simulink model "Inverter_book"  (R2025a)
settings: Solver=VariableStepAuto  StartTime=0.0  StopTime=0.1  RelTol=1e-3
libraries: spsSeriesRLCBranchLib x5, spsCurrentMeasurementLib x4, spsDiodeLib x4, spsMosfetLib x4, spsVoltageMeasurementLib x4, spsDCVoltageSourceLib x1, spsMutualInductanceLib x1, spspowerguiLib x1
settings Model: Creator=Admin  LastModifiedBy=Athip

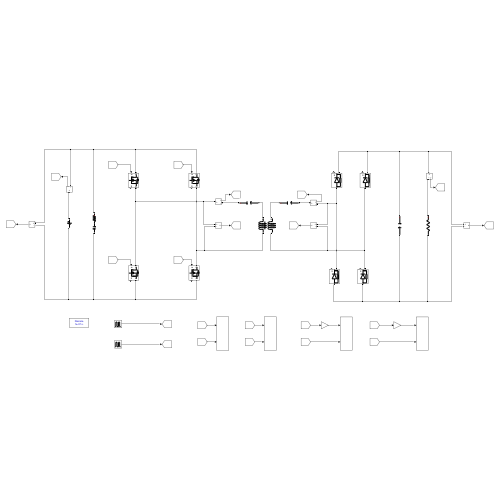
[thumbnail: Simulink's stored preview of the top-level diagram]
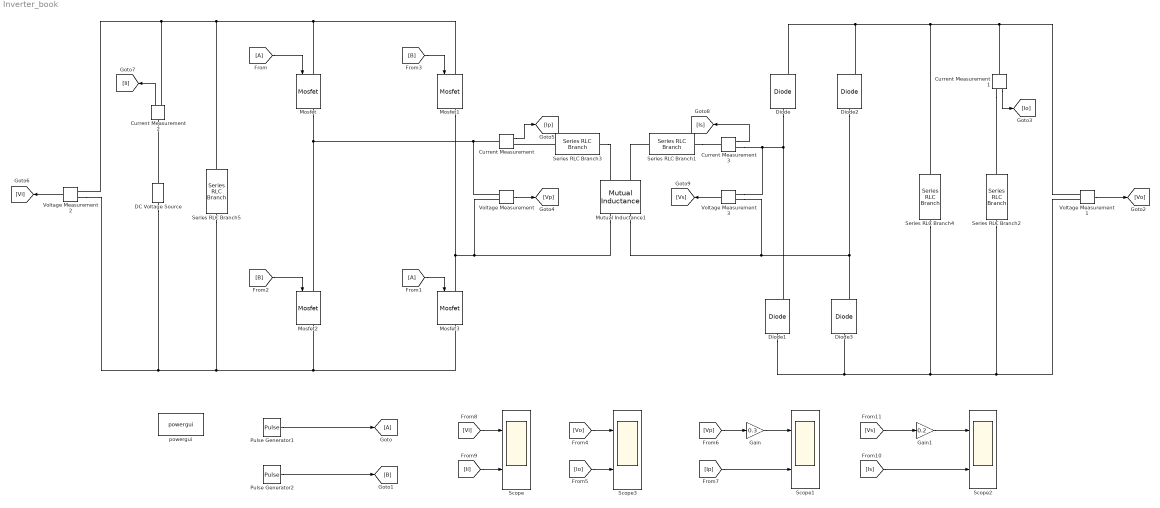
== system Inverter_book ==
  Current Measurement{,1..3} (4 alike) : spsCurrentMeasurementLib/Current Measurement  PhasorSimulation=off  OutputType=Complex  PSBequivalent=0
  DC Voltage Source : spsDCVoltageSourceLib/DC Voltage Source  Amplitude=10  Measurements=None
  Diode{,1..3} (4 alike) : spsDiodeLib/Diode  Ron=0.001  Lon=0  Vf=0.45  IC=0  UseSnubber=0  Rs=500  Cs=250e-9  Measurements=on
  From : From
  From1 : From
  Gain : Gain  Gain=0.3
  Gain1 : Gain  Gain=0.2
  Goto : Goto
  Mosfet{,1..3} (4 alike) : spsMosfetLib/Mosfet  Ron=0.0175  Lon=0  Rd=0.01  Vfd=0  IC=0  Rs=1e5  Cs=inf  Measurements=on
  Mutual Inductance1 : spsMutualInductanceLib/Mutual Inductance  LConnTagsString=a|b  RConnTagsString=A|B  TypeOfMutual=Two or three windings with equal mutual terms  NumberOfWindings=3  SelfImpedance1=[520.266e-3 16.7529e-6]  SelfImpedance2=[508.686e-3 16.0486e-6]  ThreeWindings=off  SelfImpedance3=[ 1.1 1.1e-03]  MutualImpedance=[0 7.19e-6]  InductanceMatrix="[1.0 0.9  0.9 ;  0.9 1.0  0.9;  0.9 0.9 1.0 ] * 1e-3"  ResistanceMatrix="[1.0 0.9  0.9 ;  0.9 1.0  0.9;  0.9 0.9 1.0 ]"  Measurements=None
      settings: LibrarySourceBlock=sps_lib/Passives/Mutual Inductance
  Pulse Generator1 : DiscretePulseGenerator  PulseType=Time based  Amplitude=15  Period=11.76e-6  PulseWidth=47.87
  Pulse Generator2 : DiscretePulseGenerator  PulseType=Time based  Amplitude=15  Period=11.76e-6  PulseWidth=47.87  PhaseDelay=11.76e-6/2
  Scope{,1..3} (4 alike) : Scope  NumInputPorts=2
      Scope settings: ActiveDisplayYMinimum=9  ActiveDisplayYMaximum=11
      Scope1 settings: ActiveDisplayYMinimum=-1.3979646704060489  ActiveDisplayYMaximum=4.2255749021124185
      Scope3 settings: ActiveDisplayYMinimum=0  ActiveDisplayYMaximum=18
  Series RLC Branch1 : spsSeriesRLCBranchLib/Series RLC Branch  LConnTagsString=__new0  RConnTagsString=__new0  BranchType=C  Resistance=1  Inductance=1e-3  SetiL0=off  InitialCurrent=0  Capacitance=216.1e-9  Setx0=off  InitialVoltage=0  Measurements=None
  Series RLC Branch2 : spsSeriesRLCBranchLib/Series RLC Branch  LConnTagsString=__new0  RConnTagsString=__new0  BranchType=R  Resistance=10  Inductance=1e-3  SetiL0=off  InitialCurrent=0  Capacitance=188.795e-9  Setx0=off  InitialVoltage=0  Measurements=None
  Series RLC Branch3 : spsSeriesRLCBranchLib/Series RLC Branch  LConnTagsString=__new0  RConnTagsString=__new0  BranchType=C  Resistance=1  Inductance=1e-3  SetiL0=off  InitialCurrent=0  Capacitance=214.4e-9  Setx0=off  InitialVoltage=0  Measurements=None
  Series RLC Branch4 : spsSeriesRLCBranchLib/Series RLC Branch  LConnTagsString=__new0  RConnTagsString=__new0  BranchType=C  Resistance=1  Inductance=1e-3  SetiL0=off  InitialCurrent=0  Capacitance=470e-6  Setx0=off  InitialVoltage=0  Measurements=None
  Series RLC Branch5 : spsSeriesRLCBranchLib/Series RLC Branch  LConnTagsString=__new0  RConnTagsString=__new0  BranchType=RC  Resistance=0.001  Inductance=1e-3  SetiL0=off  InitialCurrent=0  Capacitance=660e-6  Setx0=off  InitialVoltage=0  Measurements=None
  Voltage Measurement{,1..3} (4 alike) : spsVoltageMeasurementLib/Voltage Measurement  PhasorSimulation=off  OutputType=Complex  PSBequivalent=0
  powergui : spspowerguiLib/powergui  Priority=1  SimulationMode=Discrete  SampleTime=1e-7  frequency=60  Iterations=50  frequencyindice=0  Pbase=100e6  ErrMax=1e-4  UnitsV=kV  UnitsW=MW  buscounter=0  FunctionMessages=off  echomessages=off  EnableUseOfTLC=off  CurrentSourceSwitches=off  DisableSnubberDevices=off  DisableRonSwitches=off  DisableVfSwitches=off  DisplayEquations=off  AutomaticDiscreteSolvers=off  SolverType=Tustin/Backward Euler (TBE)  Interpol=off  ExternalGateDelay=off  methode=off  Ts=100  x0status=blocks  SPID=on  SwTol=0  HookPort=off  NonlinearTolerance=1e-4  nMaxIteration=100  ContinueOnMaxIteration=off  RestoreLinks=warning  ResistiveCurrentMeasurement=off  Frange=[0:2:500]  Ylog=off  Xlog=on  ShowGrid=off  save=off  variable=ZData  structure=0  ZoomFFT=off  StartTime=0.0  cycles=1  DisplayStyle=1  fundamental=60  FreqAxis=off  MaxFrequency=1000  frequencyindicesteady=1  RmsSteady=1  display=off
  wires:
  Pulse Generator1/1 -> Goto/1
  From/1 -> Mosfet/1
  From1/1 -> Mosfet3/1
  [B] -> Mosfet2/1
  [B] -> Mosfet1/1
  Voltage Measurement/1 -> [Vp]
  Current Measurement/1 -> [Ip]
  Pulse Generator2/1 -> [B]
  Voltage Measurement1/1 -> [Vo]
  Current Measurement1/1 -> [Io]
  Voltage Measurement2/1 -> [Vi]
  Current Measurement2/1 -> [Ii]
  [Vi] -> Scope/1
  [Ii] -> Scope/2
  [Ip] -> Scope1/2
  Current Measurement3/1 -> [Is]
  Voltage Measurement3/1 -> [Vs]
  [Is] -> Scope2/2
  [Vp] -> Gain/1
  Gain/1 -> Scope1/1
  [Vs] -> Gain1/1
  Gain1/1 -> Scope2/1
  [Vo] -> Scope3/1
  [Io] -> Scope3/2
  connections:
  Mosfet/RConn1 -- Voltage Measurement/LConn1 -- Current Measurement/LConn1 -- Mosfet2/LConn1
  Mosfet1/RConn1 -- Mutual Inductance1/RConn1 -- Voltage Measurement/LConn2 -- Mosfet3/LConn1
  Mosfet/LConn1 -- Mosfet1/LConn1 -- Current Measurement2/RConn1 -- Voltage Measurement2/LConn1 -- Series RLC Branch5/LConn1
  DC Voltage Source/LConn1 -- Voltage Measurement2/LConn2 -- Series RLC Branch5/RConn1 -- Mosfet3/RConn1 -- Mosfet2/RConn1
  Series RLC Branch1/LConn1 -- Mutual Inductance1/LConn2
  Series RLC Branch3/LConn1 -- Current Measurement/RConn1
  Series RLC Branch3/RConn1 -- Mutual Inductance1/LConn1
  Diode/LConn1 -- Current Measurement3/RConn1 -- Voltage Measurement3/LConn1 -- Diode1/RConn1
  Diode2/LConn1 -- Mutual Inductance1/RConn2 -- Voltage Measurement3/LConn2 -- Diode3/RConn1
  Diode2/RConn1 -- Current Measurement1/LConn1 -- Voltage Measurement1/LConn1 -- Series RLC Branch4/LConn1 -- Diode/RConn1
  Diode1/LConn1 -- Series RLC Branch2/RConn1 -- Voltage Measurement1/LConn2 -- Series RLC Branch4/RConn1 -- Diode3/LConn1
  Current Measurement1/RConn1 -- Series RLC Branch2/LConn1
  DC Voltage Source/RConn1 -- Current Measurement2/LConn1
  Series RLC Branch1/RConn1 -- Current Measurement3/LConn1
